simulink model "finalmodel1"  (R2024b)
settings: Solver=FixedStepDiscrete  StartTime=0.0  StopTime=110  FixedStep=SampleTime  MaxStep=1e-3  RelTol=1e-4  AbsTol=1e-3
InitFcn:
  | Ts=50e-6; SampleTime=50e-6; PSSMODEL=1;
  | MB=[1   0.2 30   1.25 40    12 160];
  | 
  | k=[8.3222    2.6014   19.0811    1.9818    3.6841   19.1783  240.6785    2.5684    4.3666   58.7391 7.6960   47.7975    8.7139  296.2463    2.7543    6.5051   47.7755    0.4780   35.4950   18.1866 94.2186]
  | k1=k(1);
  | k2=k(2);
  | k3=k(3);
  | k4=k(4);
  | k5=k(5);
  | k6=k(6);
  | k7=k(7);
  | k8=k(8);
  | k9=k(9);
  | k10=k(10);
  | k11=k(11);
  | k12=k(12);
  | k13=k(13);
  | k14=k(14);
  | k15=k(15);
  | k16=k(16);
  | k17=k(17);
  | k18=k(18);
  | k19=k(19);
  | k20=k(20);
  | k21=k(21);
undefined symbols (not defined in the file or in its folder): dEgdT, DiscIntNeverNeededParam, EgRef, gcbh, Rsh_array5pc, sigbuilder_block, sps_rtmsupport, Tref_K, VT_ref
libraries: spsThreePhaseVIMeasurementLib x14, spsLoadFlowBusLib x9, spsThreePhasePISectionLineLib x6, spsSeriesRLCBranchLib x5, spsThreePhaseTransformerTwoWindingsLib x4, slpidlib x4, spsThreePhaseParallelRLCLoadLib x4, spsThreePhaseSeriesRLCBranchLib x3, spsAlphaBetaZerotodq0Lib x2, spsSynchronousMachinepuStandardLib x2, spsExcitationSystemLib x2, spsMultiBandPowerSystemStabilizerLib x2
(part 8 of 9)

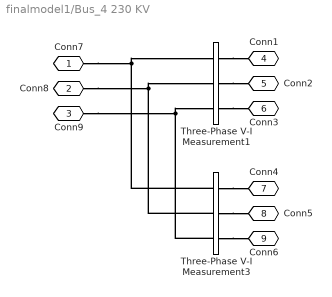
== system finalmodel1/Bus_4 230 KV ==
  Three-Phase V-I Measurement1 : spsThreePhaseVIMeasurementLib/Three-Phase V-I Measurement  VoltageMeasurement=phase-to-ground  SetLabelV=on  LabelV=Vabc_45  Vpu=on  VpuLL=off  CurrentMeasurement=yes  SetLabelI=on  LabelI=Iabc_45  Ipu=on  Pbase=100e6  Vbase=230e3  OutputType=Complex  PhasorSimulation=off  PSBequivalent=0
  Three-Phase V-I Measurement3 : spsThreePhaseVIMeasurementLib/Three-Phase V-I Measurement  VoltageMeasurement=phase-to-ground  SetLabelV=on  LabelV=Vabc_46  Vpu=on  VpuLL=off  CurrentMeasurement=yes  SetLabelI=on  LabelI=Iabc_46  Ipu=on  Pbase=100e6  Vbase=230e3  OutputType=Complex  PhasorSimulation=off  PSBequivalent=0
  Conn7 : PMIOPort  Side=Left  SampleTime=SampleTime
  Conn8 : PMIOPort  Port=2  Side=Left  SampleTime=SampleTime
  Conn9 : PMIOPort  Port=3  Side=Left  SampleTime=SampleTime
  Conn1 : PMIOPort  Port=4  Side=Right  SampleTime=SampleTime
  Conn2 : PMIOPort  Port=5  Side=Right  SampleTime=SampleTime
  Conn3 : PMIOPort  Port=6  Side=Right  SampleTime=SampleTime
  Conn4 : PMIOPort  Port=7  Side=Right  SampleTime=SampleTime
  Conn5 : PMIOPort  Port=8  Side=Right  SampleTime=SampleTime
  Conn6 : PMIOPort  Port=9  Side=Right  SampleTime=SampleTime
  connections:
  Three-Phase V-I Measurement3/LConn3 -- Conn9/RConn1 -- Three-Phase V-I Measurement1/LConn3
  Three-Phase V-I Measurement3/LConn2 -- Conn8/RConn1 -- Three-Phase V-I Measurement1/LConn2
  Three-Phase V-I Measurement3/LConn1 -- Conn7/RConn1 -- Three-Phase V-I Measurement1/LConn1
  Three-Phase V-I Measurement3/RConn3 -- Conn6/RConn1
  Three-Phase V-I Measurement1/RConn3 -- Conn3/RConn1
  Three-Phase V-I Measurement1/RConn1 -- Conn1/RConn1
  Three-Phase V-I Measurement1/RConn2 -- Conn2/RConn1
  Three-Phase V-I Measurement3/RConn1 -- Conn4/RConn1
  Three-Phase V-I Measurement3/RConn2 -- Conn5/RConn1

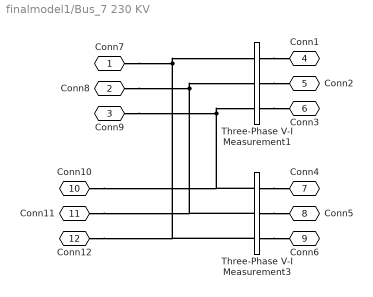
== system finalmodel1/Bus_7 230 KV ==
  Three-Phase V-I Measurement1 : spsThreePhaseVIMeasurementLib/Three-Phase V-I Measurement  VoltageMeasurement=phase-to-ground  SetLabelV=on  LabelV=Vabc_7  Vpu=on  VpuLL=off  CurrentMeasurement=yes  SetLabelI=on  LabelI=Iabc_7  Ipu=on  Pbase=100e6  Vbase=230e3  OutputType=Complex  PhasorSimulation=off  PSBequivalent=0
  Three-Phase V-I Measurement3 : spsThreePhaseVIMeasurementLib/Three-Phase V-I Measurement  VoltageMeasurement=phase-to-ground  SetLabelV=on  LabelV=Vab  Vpu=on  VpuLL=off  CurrentMeasurement=yes  SetLabelI=on  LabelI=Iab  Ipu=on  Pbase=100e6  Vbase=230e3  OutputType=Complex  PhasorSimulation=off  PSBequivalent=0
  Conn7 : PMIOPort  Side=Left  SampleTime=SampleTime
  Conn8 : PMIOPort  Port=2  Side=Left  SampleTime=SampleTime
  Conn9 : PMIOPort  Port=3  Side=Left  SampleTime=SampleTime
  Conn1 : PMIOPort  Port=4  Side=Right  SampleTime=SampleTime
  Conn2 : PMIOPort  Port=5  Side=Right  SampleTime=SampleTime
  Conn3 : PMIOPort  Port=6  Side=Right  SampleTime=SampleTime
  Conn4 : PMIOPort  Port=7  Side=Right  SampleTime=SampleTime
  Conn5 : PMIOPort  Port=8  Side=Right  SampleTime=SampleTime
  Conn6 : PMIOPort  Port=9  Side=Right  SampleTime=SampleTime
  Conn10 : PMIOPort  Port=10  Side=Left  SampleTime=SampleTime
  Conn11 : PMIOPort  Port=11  Side=Left  SampleTime=SampleTime
  Conn12 : PMIOPort  Port=12  Side=Left  SampleTime=SampleTime
  connections:
  Three-Phase V-I Measurement3/RConn2 -- Conn5/RConn1
  Three-Phase V-I Measurement3/RConn1 -- Conn4/RConn1
  Three-Phase V-I Measurement1/RConn2 -- Conn2/RConn1
  Three-Phase V-I Measurement1/RConn1 -- Conn1/RConn1
  Three-Phase V-I Measurement1/RConn3 -- Conn3/RConn1
  Three-Phase V-I Measurement3/RConn3 -- Conn6/RConn1
  Conn7/RConn1 -- Three-Phase V-I Measurement3/LConn3 -- Conn12/RConn1 -- Three-Phase V-I Measurement1/LConn1
  Conn8/RConn1 -- Three-Phase V-I Measurement3/LConn2 -- Conn11/RConn1 -- Three-Phase V-I Measurement1/LConn2
  Conn9/RConn1 -- Conn10/RConn1 -- Three-Phase V-I Measurement3/LConn1 -- Three-Phase V-I Measurement1/LConn3

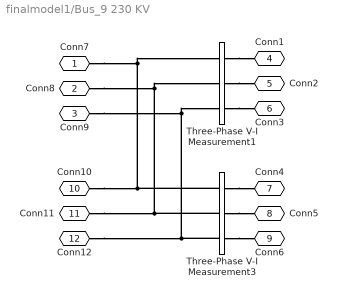
== system finalmodel1/Bus_9 230 KV ==
  Three-Phase V-I Measurement1 : spsThreePhaseVIMeasurementLib/Three-Phase V-I Measurement  VoltageMeasurement=phase-to-ground  SetLabelV=on  LabelV=Vabc_9  Vpu=on  VpuLL=off  CurrentMeasurement=yes  SetLabelI=on  LabelI=Iabc_9  Ipu=on  Pbase=100e6  Vbase=230e3  OutputType=Complex  PhasorSimulation=off  PSBequivalent=0
  Three-Phase V-I Measurement3 : spsThreePhaseVIMeasurementLib/Three-Phase V-I Measurement  VoltageMeasurement=phase-to-ground  SetLabelV=on  LabelV=Vabc  Vpu=on  VpuLL=off  CurrentMeasurement=yes  SetLabelI=on  LabelI=Iabc  Ipu=on  Pbase=100e6  Vbase=230e3  OutputType=Complex  PhasorSimulation=off  PSBequivalent=0
  Conn7 : PMIOPort  Side=Left  SampleTime=SampleTime
  Conn8 : PMIOPort  Port=2  Side=Left  SampleTime=SampleTime
  Conn9 : PMIOPort  Port=3  Side=Left  SampleTime=SampleTime
  Conn1 : PMIOPort  Port=4  Side=Right  SampleTime=SampleTime
  Conn2 : PMIOPort  Port=5  Side=Right  SampleTime=SampleTime
  Conn3 : PMIOPort  Port=6  Side=Right  SampleTime=SampleTime
  Conn4 : PMIOPort  Port=7  Side=Right  SampleTime=SampleTime
  Conn5 : PMIOPort  Port=8  Side=Right  SampleTime=SampleTime
  Conn6 : PMIOPort  Port=9  Side=Right  SampleTime=SampleTime
  Conn10 : PMIOPort  Port=10  Side=Left  SampleTime=SampleTime
  Conn11 : PMIOPort  Port=11  Side=Left  SampleTime=SampleTime
  Conn12 : PMIOPort  Port=12  Side=Left  SampleTime=SampleTime
  connections:
  Conn12/RConn1 -- Three-Phase V-I Measurement3/LConn3 -- Conn9/RConn1 -- Three-Phase V-I Measurement1/LConn3
  Conn11/RConn1 -- Three-Phase V-I Measurement3/LConn2 -- Conn8/RConn1 -- Three-Phase V-I Measurement1/LConn2
  Conn10/RConn1 -- Three-Phase V-I Measurement3/LConn1 -- Conn7/RConn1 -- Three-Phase V-I Measurement1/LConn1
  Three-Phase V-I Measurement3/RConn3 -- Conn6/RConn1
  Three-Phase V-I Measurement1/RConn3 -- Conn3/RConn1
  Three-Phase V-I Measurement1/RConn1 -- Conn1/RConn1
  Three-Phase V-I Measurement1/RConn2 -- Conn2/RConn1
  Three-Phase V-I Measurement3/RConn1 -- Conn4/RConn1
  Three-Phase V-I Measurement3/RConn2 -- Conn5/RConn1

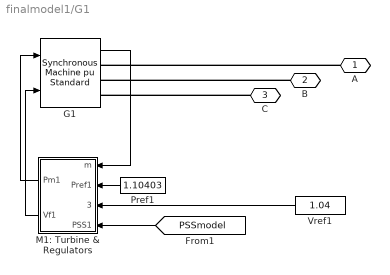
== system finalmodel1/G1 ==
  G1 : spsSynchronousMachinepuStandardLib/Synchronous Machine pu Standard  PresetModel=No  MechanicalLoad=Mechanical power Pm  ShowDetailedParameters=on  RotorType=Round  Units=per unit standard parameters  MeasurementBus=off  NominalParameters="[247.5e6  16500   60 ]"  Reactances1=[1.146 0.2998 0.25 0.969 0.45 0.25 0.025]  Reactances2=[ 1.305, 0.296, 0.252, 0.474, 0.243, 0.18 ]  dAxisTimeConstants=Open-circuit  qAxisTimeConstants=Open-circuit  TimeConstants1=[]  TimeConstants2=[8.96 0.05 0.31 0.05]  TimeConstants3=[]  TimeConstants4=[]  TimeConstants5=[ 1.01, 0.053, 0.1 ]  TimeConstants6=[]  TimeConstants7=[]  TimeConstants8=[]  StatorResistance=0.0025  Mechanical="[ 23.64  0  4]"  PolePairs=4  InitialConditions=[0 -52.9545 0.924925 0.924925 0.924925 -8.45401 -128.454 111.546 1.58772]  SetSaturation=off  Saturation=[0.6404,0.7127,0.8441,0.9214,0.9956,1.082,1.19,1.316,1.457;0.7,0.7698,0.8872,0.9466,0.9969,1.046,1.1,1.151,1.201]  LoadFlowParameters=[2 128000000 0 0 0]  TsPowergui=0  TsBlock=-1  IterativeModel=Trapezoidal non iterative  IterativeDiscreteModel=Trapezoidal non iterative  BusType=swing  Pref=NaN  Qref=0  Qmin=-Inf  Qmax=Inf  PLF=0  QLF=0
      link override Electrical model/Synchronous Machine Discrete Model/Saturation/Lmd_sat/Lmd_sat: SampleTime=SampleTime
      link override Electrical model/Synchronous Machine Discrete Model/Saturation/Lmq_sat/Lmq_sat: SampleTime=SampleTime
      link override Electrical model/Synchronous Machine Discrete Model/phi/Digital Clock: SampleTime=SampleTime
      link override Electrical model/Synchronous Machine Discrete Model/phi/fluxes: SampleTime=SampleTime
      link override Electrical model/Synchronous Machine Discrete Model/phi/voltages: SampleTime=SampleTime
      link override Mechanical model/Delay Prediction/dw_delay: SampleTime=SampleTime
      link override Mechanical model/Delay Prediction/dw_predict: SampleTime=SampleTime
      link override Mechanical model/Digital Clock: SampleTime=SampleTime
      link override Mechanical model/Fcn: Expr=rem(u,2*pi)
      link override Mechanical model/Rotor angle dthetae: SampleTime=SampleTime
      link override Mechanical model/Rotor speed deviation (dw): SampleTime=SampleTime
      link override Mechanical model/theta: SampleTime=SampleTime
  M1: Turbine & Regulators : Subsystem
  Pref1 : Constant  Value=1.10403  SampleTime=SampleTime
  Vref1 : Constant  Value=1.04  SampleTime=SampleTime
  A : PMIOPort  Side=Left  SampleTime=SampleTime
  B : PMIOPort  Port=2  Side=Left  SampleTime=SampleTime
  C : PMIOPort  Port=3  Side=Left  SampleTime=SampleTime
  wires:
  Pref1/1 -> M1: Turbine & Regulators/2(Pref1)
  [PSSmodel] -> M1: Turbine & Regulators/4(PSS1)
  M1: Turbine & Regulators/1(Pm1) -> G1/1
  M1: Turbine & Regulators/2(Vf1) -> G1/2
  G1/1 -> M1: Turbine & Regulators/1(m)
  Vref1/1 -> M1: Turbine & Regulators/3(Vref1)
  connections:
  A/RConn1 -- G1/RConn1
  B/RConn1 -- G1/RConn2
  C/RConn1 -- G1/RConn3

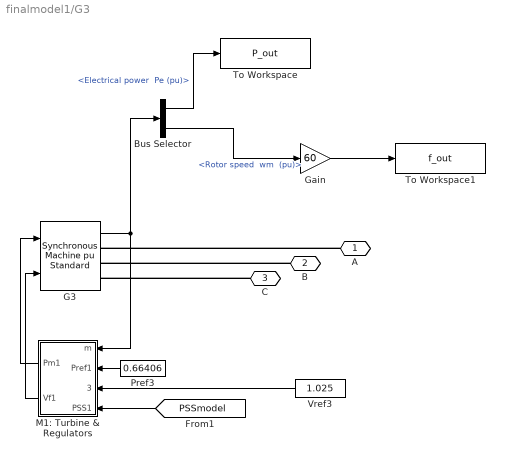
== system finalmodel1/G3 ==
  Bus Selector : BusSelector  OutputSignals="Mechanical.Electrical power  Pe (pu),Mechanical.Rotor speed  wm  (pu)"
  G3 : spsSynchronousMachinepuStandardLib/Synchronous Machine pu Standard  PresetModel=No  MechanicalLoad=Mechanical power Pm  ShowDetailedParameters=on  RotorType=Round  Units=per unit standard parameters  MeasurementBus=off  NominalParameters="[128e6  13800   60 ]"  Reactances1=[1.3125 0.2998 0.25 1.2578 0.45 0.25 0.025]  Reactances2=[ 1.305, 0.296, 0.252, 0.474, 0.243, 0.18 ]  dAxisTimeConstants=Open-circuit  qAxisTimeConstants=Open-circuit  TimeConstants1=[]  TimeConstants2=[5.89 0.05 0.6 0.05]  TimeConstants3=[]  TimeConstants4=[]  TimeConstants5=[ 1.01, 0.053, 0.1 ]  TimeConstants6=[]  TimeConstants7=[]  TimeConstants8=[]  StatorResistance=0.0025  Mechanical="[ 3.01  0  4]"  PolePairs=4  InitialConditions=[0 -58.3097 0.651492 0.651492 0.651492 -3.18103 -123.181 116.819 1.26474]  SetSaturation=off  Saturation=[0.6404,0.7127,0.8441,0.9214,0.9956,1.082,1.19,1.316,1.457;0.7,0.7698,0.8872,0.9466,0.9969,1.046,1.1,1.151,1.201]  LoadFlowParameters=[1 85000000 0 0 0]  TsPowergui=0  TsBlock=-1  IterativeModel=Trapezoidal non iterative  IterativeDiscreteModel=Trapezoidal non iterative  BusType=PV  Pref=85e6  Qref=0  Qmin=-Inf  Qmax=Inf  PLF=0  QLF=0
      link override Electrical model/Synchronous Machine Discrete Model/Saturation/Lmd_sat/Lmd_sat: SampleTime=SampleTime
      link override Electrical model/Synchronous Machine Discrete Model/Saturation/Lmq_sat/Lmq_sat: SampleTime=SampleTime
      link override Electrical model/Synchronous Machine Discrete Model/phi/Digital Clock: SampleTime=SampleTime
      link override Electrical model/Synchronous Machine Discrete Model/phi/fluxes: SampleTime=SampleTime
      link override Electrical model/Synchronous Machine Discrete Model/phi/voltages: SampleTime=SampleTime
      link override Mechanical model/Delay Prediction/dw_delay: SampleTime=SampleTime
      link override Mechanical model/Delay Prediction/dw_predict: SampleTime=SampleTime
      link override Mechanical model/Digital Clock: SampleTime=SampleTime
      link override Mechanical model/Fcn: Expr=rem(u,2*pi)
      link override Mechanical model/Rotor angle dthetae: SampleTime=SampleTime
      link override Mechanical model/Rotor speed deviation (dw): SampleTime=SampleTime
      link override Mechanical model/theta: SampleTime=SampleTime
  Gain : Gain  Gain=60  SampleTime=SampleTime
  M1: Turbine & Regulators : Subsystem
  Pref3 : Constant  Value=0.66406  SampleTime=SampleTime
  To Workspace : ToWorkspace  VariableName=P_out  SaveFormat=Timeseries  SampleTime=SampleTime
  To Workspace1 : ToWorkspace  VariableName=f_out  SaveFormat=Timeseries  SampleTime=SampleTime
  Vref3 : Constant  Value=1.025  SampleTime=SampleTime
  A : PMIOPort  Side=Left  SampleTime=SampleTime
  B : PMIOPort  Port=2  Side=Left  SampleTime=SampleTime
  C : PMIOPort  Port=3  Side=Left  SampleTime=SampleTime
  wires:
  Vref3/1 -> M1: Turbine & Regulators/3(Vref1)
  G3/1 -> Bus Selector/1, M1: Turbine & Regulators/1(m)
  M1: Turbine & Regulators/2(Vf1) -> G3/2
  M1: Turbine & Regulators/1(Pm1) -> G3/1
  [PSSmodel] -> M1: Turbine & Regulators/4(PSS1)
  Pref3/1 -> M1: Turbine & Regulators/2(Pref1)
  Gain/1 -> To Workspace1/1
  Bus Selector/1 -> To Workspace/1  "<Electrical power  Pe (pu)>"
  Bus Selector/2 -> Gain/1  "<Rotor speed  wm  (pu)>"
  connections:
  C/RConn1 -- G3/RConn3
  B/RConn1 -- G3/RConn2
  A/RConn1 -- G3/RConn1

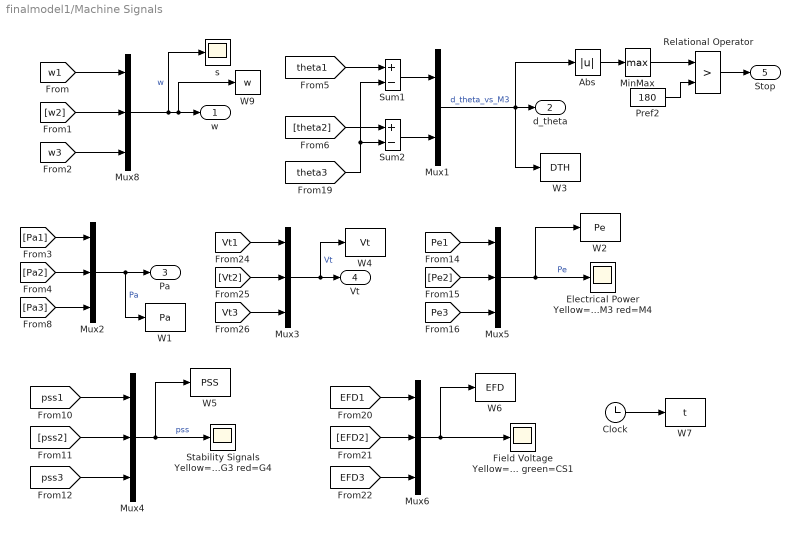
== system finalmodel1/Machine Signals ==
  Abs : Abs  SampleTime=SampleTime
  Clock : Clock
  "Electrical Power Yellow=M1 mag=M2 cyan=M3 red=M4 " : Scope
  Field Voltage Yellow=G1 mag=G2 cyan=G3 red=G4 green=CS1 : Scope
  MinMax : MinMax  Function=max  InputSameDT=on  SaturateOnIntegerOverflow=on  SampleTime=SampleTime
  Mux1 : Mux  Inputs=2
  Mux{2..6,8} (6 alike) : Mux  Inputs=3
  Pref2 : Constant  Value=180  SampleTime=SampleTime
  Relational Operator : RelationalOperator  Operator=>  SampleTime=SampleTime
  "Stability Signals Yellow=G1 mag=G2 cyan=G3 red=G4 " : Scope
  Sum1 : Sum  Inputs=+-  InputSameDT=on  SaturateOnIntegerOverflow=on  SampleTime=SampleTime  OutDataTypeStr=Inherit: Same as first input
  Sum2 : Sum  Inputs=+-  InputSameDT=on  SaturateOnIntegerOverflow=on  SampleTime=SampleTime  OutDataTypeStr=Inherit: Same as first input
  W1 : ToWorkspace  VariableName=Pa  SaveFormat=Timeseries  SampleTime=SampleTime
  W2 : ToWorkspace  VariableName=Pe  SaveFormat=Timeseries  SampleTime=SampleTime
  W3 : ToWorkspace  VariableName=DTH  SaveFormat=Timeseries  SampleTime=SampleTime
  W4 : ToWorkspace  VariableName=Vt  SaveFormat=Timeseries  SampleTime=SampleTime
  W5 : ToWorkspace  VariableName=PSS  SaveFormat=Timeseries  SampleTime=SampleTime
  W6 : ToWorkspace  VariableName=EFD  SaveFormat=Timeseries  SampleTime=SampleTime
  W7 : ToWorkspace  VariableName=t  SaveFormat=Timeseries  SampleTime=SampleTime
  W9 : ToWorkspace  VariableName=w  SaveFormat=Timeseries  SampleTime=SampleTime
  s : Scope
  w : Outport  SampleTime=SampleTime
  d_theta : Outport  Port=2  SampleTime=SampleTime
  Pa : Outport  Port=3  SampleTime=SampleTime
  Vt : Outport  Port=4  SampleTime=SampleTime
  Stop : Outport  Port=5  SampleTime=SampleTime
  wires:
  Mux8/1 -> s/1, W9/1, w/1  "w"
  [w1] -> Mux8/1
  [w2] -> Mux8/2
  [w3] -> Mux8/3
  Mux1/1 -> d_theta/1, Abs/1, W3/1  "d_theta_vs_M3"
  Abs/1 -> MinMax/1
  Pref2/1 -> Relational Operator/2
  MinMax/1 -> Relational Operator/1
  [Pa1] -> Mux2/1
  Mux4/1 -> "Stability Signals Yellow=G1 mag=G2 cyan=G3 red=G4 "/1, W5/1  "pss"
  [pss1] -> Mux4/1
  [pss2] -> Mux4/2
  [pss3] -> Mux4/3
  [EFD1] -> Mux6/1
  [EFD2] -> Mux6/2
  [EFD3] -> Mux6/3
  Mux6/1 -> Field Voltage Yellow=G1 mag=G2 cyan=G3 red=G4 green=CS1/1, W6/1
  Relational Operator/1 -> Stop/1
  Mux2/1 -> Pa/1, W1/1  "Pa"
  [theta1] -> Sum1/1
  Sum1/1 -> Mux1/1
  [theta2] -> Sum2/1
  [theta3] -> Sum1/2, Sum2/2
  Sum2/1 -> Mux1/2
  [Pa2] -> Mux2/2
  [Pa3] -> Mux2/3
  [Vt1] -> Mux3/1
  [Vt2] -> Mux3/2
  [Vt3] -> Mux3/3
  Mux3/1 -> Vt/1, W4/1  "Vt"
  [Pe1] -> Mux5/1
  [Pe2] -> Mux5/2
  [Pe3] -> Mux5/3
  Mux5/1 -> "Electrical Power Yellow=M1 mag=M2 cyan=M3 red=M4 "/1, W2/1  "Pe"
  Clock/1 -> W7/1

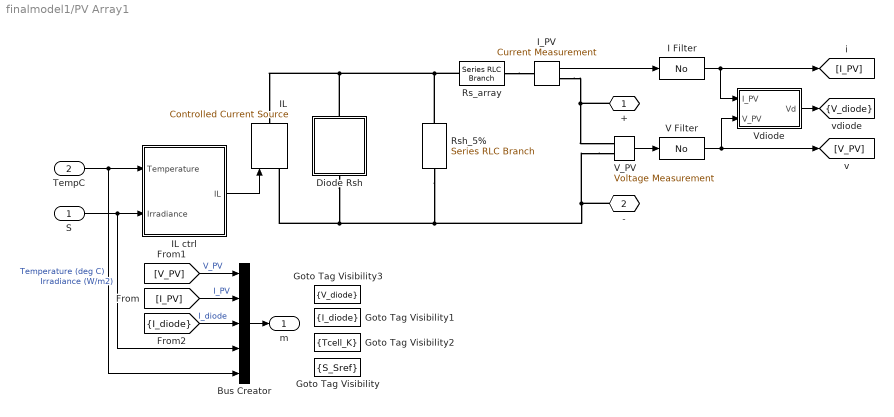
== system finalmodel1/PV Array1 ==
  S : Inport
  TempC : Inport  Port=2
  Bus Creator : BusCreator  Inputs=5
  Diode Rsh : Subsystem
      mask Display:
      | plot(-75,-50,100,150, [-15 -15 43 -15 -15 -75],[50 8 50 92 50 50], ...
      |     [43 43],[8 94],[100 43], [50 50])
  Goto Tag Visibility : GotoTagVisibility  GotoTag=S_Sref
  Goto Tag Visibility1 : GotoTagVisibility  GotoTag=I_diode
  Goto Tag Visibility2 : GotoTagVisibility  GotoTag=Tcell_K
  Goto Tag Visibility3 : GotoTagVisibility  GotoTag=V_diode
  I Filter : spsPVarrayModel/No  SystemSampleTime=-1  VariantControl=Variant1  VariantActivationTime=update diagram  AllowFlexibleInterface=on  Latency=0  AutoFrameSizeCalculation=off
  IL : spsControlledCurrentSourceLib/Controlled Current Source  Initialize=on  Source_Type=AC  Amplitude=0  Phase=0  Frequency=0  Measurements=None
  IL ctrl : Subsystem
  I_PV : spsCurrentMeasurementLib/Current Measurement  PhasorSimulation=off  OutputType=Complex  PSBequivalent=0
  Rs_array : spsSeriesRLCBranchLib/Series RLC Branch  LConnTagsString=__new0  RConnTagsString=__new0  BranchType=R  Resistance=Rs*Nser/Npar  Inductance=1e-3  SetiL0=off  InitialCurrent=0  Capacitance=1e-6  Setx0=off  InitialVoltage=0  Measurements=None
  Rsh_5% : spsSeriesRLCBranchLib/Series RLC Branch  LConnTagsString=__new0  RConnTagsString=__new0  BranchType=R  Resistance=Rsh_array5pc  Inductance=1e-3  SetiL0=off  InitialCurrent=0  Capacitance=1e-6  Setx0=off  InitialVoltage=0  Measurements=None
  V Filter : spsPVarrayModel/No  SystemSampleTime=-1  VariantControl=Variant1  VariantActivationTime=update diagram  AllowFlexibleInterface=on  Latency=0  AutoFrameSizeCalculation=off
  V_PV : spsVoltageMeasurementLib/Voltage Measurement  PhasorSimulation=off  OutputType=Complex  PSBequivalent=0
  Vdiode : Subsystem
  + : PMIOPort  Side=Right
  - : PMIOPort  Port=2  Side=Right
  m : Outport  VectorParamsAs1DForOutWhenUnconnected=off
  tag scope: V_diode=scoped
  wires:
  TempC/1 -> Bus Creator/5, IL ctrl/1(Temperature)  "Temperature (deg C)"
  S/1 -> IL ctrl/2(Irradiance), Bus Creator/4  "Irradiance (W/m2)"
  I_PV/1 -> I Filter/1
  Bus Creator/1 -> m/1
  IL ctrl/1(IL) -> IL/1
  V_PV/1 -> V Filter/1
  I Filter/1 -> Vdiode/1(I_PV), [I_PV]
  V Filter/1 -> [V_PV], Vdiode/2(V_PV)
  [I_PV] -> Bus Creator/2  "I_PV"
  [V_PV] -> Bus Creator/1  "V_PV"
  [I_diode] -> Bus Creator/3  "I_diode"
  Vdiode/1(Vd) -> [V_diode]
  connections:
  +/RConn1 -- I_PV/RConn1 -- V_PV/LConn1
  Rs_array/LConn1 -- Rsh_5%/LConn1 -- Diode Rsh/LConn1 -- IL/RConn1
  V_PV/LConn2 -- Diode Rsh/RConn1 -- IL/LConn1 -- Rsh_5%/RConn1 -- -/RConn1
  Rs_array/RConn1 -- I_PV/LConn1

== system finalmodel1/Signal Builder2 ==
  Demux : Demux  Tag=STV Demux  Outputs=1
      settings: DisplayOption=none
  FromWs : FromWorkspace  Tag=STV FromWs  VariableName=tuvar
      SigBuilderData=|
      | common.afterFinalStr = 'Extrapolate'
      | common.sampleTime = 0
      | dataSet.timeRange = [0 4]
      | dataSet.name = 'Group 1'
      | sbobj.Groups.Name = 'Group 1'
      | sbobj.Groups.Signals.Name = 'Signal 1'
      | sbobj.Groups.Signals.XData = [0 0.00416233090531 0.00832466181061 0.0124869927159 0.0166493236212 0.0208116545265 0.0249739854318 0.0291363163371 0.0332986472425 0.0374609781478 0.0416233090531 0.0457856399584 ... (962 elements, 1x962)]
      | sbobj.Groups.Signals.YData = [2.47122187864 2.47122187864 2.47122187864 2.47122187864 2.47122187864 2.47122187864 2.47122187864 2.47122187864 2.47122187864 2.47121149505 2.47121149505 2.47121149505 ... (962 elements, 1x962)]
      | sbobj.Groups.TimeRange = [0 4]
  Signal 1 : Outport  Tag=STV Outport  VectorParamsAs1DForOutWhenUnconnected=off
  wires:
  FromWs/1 -> Demux/1
  Demux/1 -> Signal 1/1

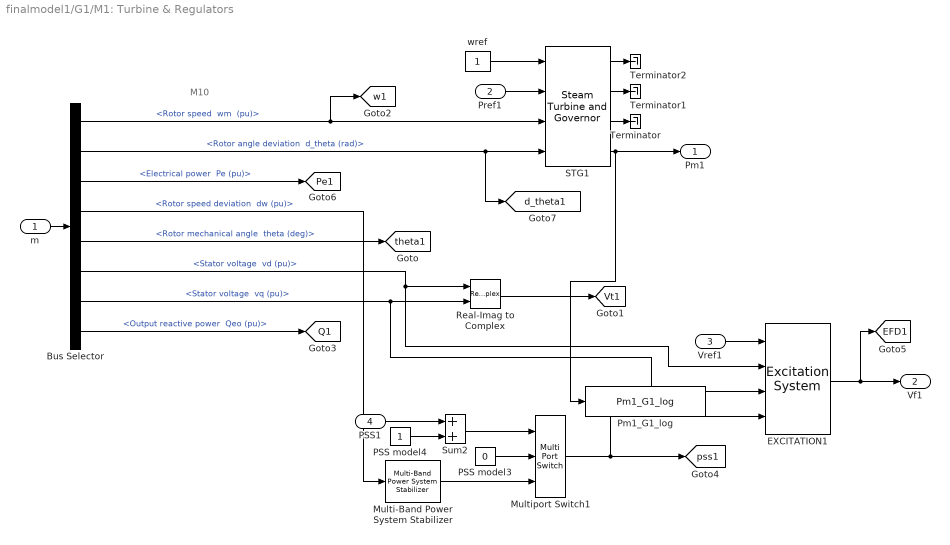
== system finalmodel1/G1/M1: Turbine & Regulators ==
  note: M10
  m : Inport  SampleTime=SampleTime
  Pref1 : Inport  Port=2  SampleTime=SampleTime
  Vref1 : Inport  Port=3  SampleTime=SampleTime
  PSS1 : Inport  Port=4  SampleTime=SampleTime
  Bus Selector : BusSelector  OutputSignals="Mechanical.Rotor speed  wm  (pu),Mechanical.Rotor angle deviation  d_theta (rad),Mechanical.Electrical power  Pe (pu),Mechanical.Rotor speed deviation  dw (pu),Mechanical.Rotor mechanical angle  theta (deg),dq0 components.Stator voltage  vd (pu),dq0 components.Stator voltage  vq (pu),Output reactive power  Qeo (pu)"
  EXCITATION1 : spsExcitationSystemLib/Excitation System  tr=0.01  reg=[20 0.2 ]  exc=[ 1, 0.314 ]  tgr=[10 1]  damp=[ 0, 0 ]  sat=[ 0, 0 ]  lim="[-5 5  0 ]"  v0=[1.04 1.5877]
      link override Model: Ts=SampleTime
      link override Model/Damping kfd.s // (tfd.s +1)/1st-Order Discrete Filter: Ts=SampleTime
      link override Model/Damping kfd.s // (tfd.s +1)/1st-Order Discrete Filter/Discrete State-Space: SampleTime=SampleTime
      link override Model/Exciter  1 // (te.s + ke)/1st order Lowpass: Ts=SampleTime
      link override Model/Exciter  1 // (te.s + ke)/1st order Lowpass/Discrete State-Space: SampleTime=SampleTime
      link override Model/Lead Lag Compensator tc.s+1 // tb.s+1: Ts=SampleTime
      link override Model/Lead Lag Compensator tc.s+1 // tb.s+1/Discrete State-Space: SampleTime=SampleTime
      link override Model/Low Pass Filter 1 // (tr.s +1) (with IC): Ts=SampleTime
      link override Model/Low Pass Filter 1 // (tr.s +1) (with IC)/Discrete State-Space: SampleTime=SampleTime
      link override Model/Main Regulator ka // (ta.s +1)/1st order Lowpass: Ts=SampleTime
      link override Model/Main Regulator ka // (ta.s +1)/1st order Lowpass/Discrete State-Space: SampleTime=SampleTime
      link override Model/Positive Sequence Voltage: Expr=sqrt(abs(u(1)^2 + u(2)^2))
      link override Model/Unit Delay1: SampleTime=SampleTime
      link override Model/Unit Delay2: SampleTime=SampleTime
      settings: LibrarySourceBlock=sps_lib/Electrical Machines/Synchronous Machine Control/Excitation System
  Multi-Band Power System Stabilizer : spsMultiBandPowerSystemStabilizerLib/Multi-Band Power System Stabilizer  OperationMode=Simplified settings  Kg=k8  GL=[k9 k10]  GI=[k11 k12]  GH=[k13 k14]  GLd=[66 66 9.4]  TcLF=[1.667 2 0 0 0 0 2 2.4 0 0 0 0 1 1]  GId=[66 66 47.6]  TcIF=[1 1 0.25 0.3 0 0 1 1 0.3 0.36 0 0 0 0]  GHd=[66 66 233]  TcHF="[0.01 0.012 0 0 0 0  0.012 0.0144 0 0 0 0 1 1]"  LIM=[.075 .15 .15 .15]  Plot_On=off  MagdB_On=off  FreqRange=logspace(-2,2,500)
      link override Model/Discrete Lead-Lag1: Ts=SampleTime
      link override Model/Discrete Lead-Lag1/Discrete State-Space: SampleTime=SampleTime
      link override Model/Discrete Lead-Lag2: Ts=SampleTime
      link override Model/Discrete Lead-Lag2/Discrete State-Space: SampleTime=SampleTime
      link override Model/Discrete Lead-Lag3: Ts=SampleTime
      link override Model/Discrete Lead-Lag3/Discrete State-Space: SampleTime=SampleTime
      link override Model/Discrete Lead-Lag4: Ts=SampleTime
      link override Model/Discrete Lead-Lag4/Discrete State-Space: SampleTime=SampleTime
      link override Model/Discrete Lead-Lag5: Ts=SampleTime
      link override Model/Discrete Lead-Lag5/Discrete State-Space: SampleTime=SampleTime
      link override Model/Discrete Lead-Lag6: Ts=SampleTime
      link override Model/Discrete Lead-Lag6/Discrete State-Space: SampleTime=SampleTime
      link override Model/HF speed sensor: Ts=SampleTime
      link override Model/HF speed sensor/Discrete State-Space: SampleTime=SampleTime
      link override Model/LF and IF speed sensor: Ts=SampleTime
      link override Model/LF and IF speed sensor/Discrete State-Space: SampleTime=SampleTime
      link override Model/Transfer function for detailed model (HF)/Transfer functions for detailed stabilizer/Discrete Lead-Lag1: Ts=SampleTime
      link override Model/Transfer function for detailed model (HF)/Transfer functions for detailed stabilizer/Discrete Lead-Lag1/Discrete State-Space: SampleTime=SampleTime
      link override Model/Transfer function for detailed model (HF)/Transfer functions for detailed stabilizer/Discrete Lead-Lag2: Ts=SampleTime
      link override Model/Transfer function for detailed model (HF)/Transfer functions for detailed stabilizer/Discrete Lead-Lag2/Discrete State-Space: SampleTime=SampleTime
      link override Model/Transfer function for detailed model (HF)/Transfer functions for detailed stabilizer1/Discrete Lead-Lag1: Ts=SampleTime
      link override Model/Transfer function for detailed model (HF)/Transfer functions for detailed stabilizer1/Discrete Lead-Lag1/Discrete State-Space: SampleTime=SampleTime
      link override Model/Transfer function for detailed model (HF)/Transfer functions for detailed stabilizer1/Discrete Lead-Lag2: Ts=SampleTime
      link override Model/Transfer function for detailed model (HF)/Transfer functions for detailed stabilizer1/Discrete Lead-Lag2/Discrete State-Space: SampleTime=SampleTime
      link override Model/Transfer function for detailed model (IF)/Transfer functions for detailed stabilizer/Discrete Lead-Lag1: Ts=SampleTime
      link override Model/Transfer function for detailed model (IF)/Transfer functions for detailed stabilizer/Discrete Lead-Lag1/Discrete State-Space: SampleTime=SampleTime
      link override Model/Transfer function for detailed model (IF)/Transfer functions for detailed stabilizer/Discrete Lead-Lag2: Ts=SampleTime
      link override Model/Transfer function for detailed model (IF)/Transfer functions for detailed stabilizer/Discrete Lead-Lag2/Discrete State-Space: SampleTime=SampleTime
      link override Model/Transfer function for detailed model (IF)/Transfer functions for detailed stabilizer1/Discrete Lead-Lag1: Ts=SampleTime
      link override Model/Transfer function for detailed model (IF)/Transfer functions for detailed stabilizer1/Discrete Lead-Lag1/Discrete State-Space: SampleTime=SampleTime
      link override Model/Transfer function for detailed model (IF)/Transfer functions for detailed stabilizer1/Discrete Lead-Lag2: Ts=SampleTime
      link override Model/Transfer function for detailed model (IF)/Transfer functions for detailed stabilizer1/Discrete Lead-Lag2/Discrete State-Space: SampleTime=SampleTime
      link override Model/Transfer function for detailed model (LF)/Transfer functions for detailed stabilizer/Discrete Lead-Lag1: Ts=SampleTime
      link override Model/Transfer function for detailed model (LF)/Transfer functions for detailed stabilizer/Discrete Lead-Lag1/Discrete State-Space: SampleTime=SampleTime
      link override Model/Transfer function for detailed model (LF)/Transfer functions for detailed stabilizer/Discrete Lead-Lag2: Ts=SampleTime
      link override Model/Transfer function for detailed model (LF)/Transfer functions for detailed stabilizer/Discrete Lead-Lag2/Discrete State-Space: SampleTime=SampleTime
      link override Model/Transfer function for detailed model (LF)/Transfer functions for detailed stabilizer1/Discrete Lead-Lag1: Ts=SampleTime
      link override Model/Transfer function for detailed model (LF)/Transfer functions for detailed stabilizer1/Discrete Lead-Lag1/Discrete State-Space: SampleTime=SampleTime
      link override Model/Transfer function for detailed model (LF)/Transfer functions for detailed stabilizer1/Discrete Lead-Lag2: Ts=SampleTime
      link override Model/Transfer function for detailed model (LF)/Transfer functions for detailed stabilizer1/Discrete Lead-Lag2/Discrete State-Space: SampleTime=SampleTime
      settings: LibrarySourceBlock=|
      | sps_lib/Electrical Machines/Synchronous Machine Control/Multi-Band
      | Power System Stabilizer
  Multiport Switch1 : MultiPortSwitch  Inputs=2  SampleTime=SampleTime  SaturateOnIntegerOverflow=off
  PSS model3 : Constant  Value=0  SampleTime=SampleTime
  PSS model4 : Constant  SampleTime=SampleTime
  Pm1_G1_log : ToWorkspace  VariableName=Pm1_G1_log  SaveFormat=Timeseries  SampleTime=-1
  Real-Imag to Complex : RealImagToComplex  SampleTime=SampleTime
  STG1 : spsSteamTurbineandGovernorLib/Steam Turbine and Governor  gentype=Tandem-compound (single mass)  reg1="[ 1  0.05    0 ]"  reg2="[ 0.001  0.15 ]"  reg3="[ -0.1  0.1  0  4.496 ]"  N=3600  turb1="[ 0  10   3.3   0.5   ]"  turb2="[   0   0.36    0.36   0.28   ]"  HA="[ 0.046  1.430  1.465   0.192 ]"  KA="[ 90.44  53.88  64.59   62.94  ]"  DA="[ 0.0115  0.3575  0.3663   0.0137  ]"  ini1=0.95361  ini2=[0.779316,-31.4247]
      link override Model/4 mass shaft/1 mass/Mass2: Ts=SampleTime
      link override Model/4 mass shaft/1 mass/Mass2/Ad*x(k-1): SampleTime=SampleTime
      link override Model/4 mass shaft/1 mass/Mass2/Bd*(u(k)+ u(k-1)): SampleTime=SampleTime
      link override Model/4 mass shaft/1 mass/Mass2/Delay_u: SampleTime=SampleTime
      link override Model/4 mass shaft/1 mass/Mass2/Delay_x: SampleTime=SampleTime
      link override Model/4 mass shaft/1 mass/Mass2/Digital Clock: SampleTime=SampleTime
      link override Model/4 mass shaft/1 mass/Mass2/Prediction/Unit Delay3: SampleTime=SampleTime
      link override Model/4 mass shaft/2 masses/Mass2: Ts=SampleTime
      link override Model/4 mass shaft/2 masses/Mass2/Ad*x(k-1): SampleTime=SampleTime
      link override Model/4 mass shaft/2 masses/Mass2/Bd*(u(k)+ u(k-1)): SampleTime=SampleTime
      link override Model/4 mass shaft/2 masses/Mass2/Delay_u: SampleTime=SampleTime
      link override Model/4 mass shaft/2 masses/Mass2/Delay_x: SampleTime=SampleTime
      link override Model/4 mass shaft/2 masses/Mass2/Digital Clock: SampleTime=SampleTime
      link override Model/4 mass shaft/2 masses/Mass2/Prediction/Unit Delay3: SampleTime=SampleTime
      link override Model/4 mass shaft/2 masses/Mass3: Ts=SampleTime
      link override Model/4 mass shaft/2 masses/Mass3/Ad*x(k-1): SampleTime=SampleTime
      link override Model/4 mass shaft/2 masses/Mass3/Bd*(u(k)+ u(k-1)): SampleTime=SampleTime
      link override Model/4 mass shaft/2 masses/Mass3/Delay_u: SampleTime=SampleTime
      link override Model/4 mass shaft/2 masses/Mass3/Delay_x: SampleTime=SampleTime
      link override Model/4 mass shaft/2 masses/Mass3/Digital Clock: SampleTime=SampleTime
      link override Model/4 mass shaft/2 masses/Mass3/Prediction/Unit Delay3: SampleTime=SampleTime
      link override Model/4 mass shaft/3 masses/Mass2: Ts=SampleTime
      link override Model/4 mass shaft/3 masses/Mass2/Ad*x(k-1): SampleTime=SampleTime
      link override Model/4 mass shaft/3 masses/Mass2/Bd*(u(k)+ u(k-1)): SampleTime=SampleTime
      link override Model/4 mass shaft/3 masses/Mass2/Delay_u: SampleTime=SampleTime
      link override Model/4 mass shaft/3 masses/Mass2/Delay_x: SampleTime=SampleTime
      link override Model/4 mass shaft/3 masses/Mass2/Digital Clock: SampleTime=SampleTime
      link override Model/4 mass shaft/3 masses/Mass2/Prediction/Unit Delay3: SampleTime=SampleTime
      link override Model/4 mass shaft/3 masses/Mass3: Ts=SampleTime
      link override Model/4 mass shaft/3 masses/Mass3/Ad*x(k-1): SampleTime=SampleTime
      link override Model/4 mass shaft/3 masses/Mass3/Bd*(u(k)+ u(k-1)): SampleTime=SampleTime
      link override Model/4 mass shaft/3 masses/Mass3/Delay_u: SampleTime=SampleTime
      link override Model/4 mass shaft/3 masses/Mass3/Delay_x: SampleTime=SampleTime
      link override Model/4 mass shaft/3 masses/Mass3/Digital Clock: SampleTime=SampleTime
      link override Model/4 mass shaft/3 masses/Mass3/Prediction/Unit Delay3: SampleTime=SampleTime
      link override Model/4 mass shaft/3 masses/Mass4: Ts=SampleTime
      link override Model/4 mass shaft/3 masses/Mass4/Ad*x(k-1): SampleTime=SampleTime
      link override Model/4 mass shaft/3 masses/Mass4/Bd*(u(k)+ u(k-1)): SampleTime=SampleTime
      link override Model/4 mass shaft/3 masses/Mass4/Delay_u: SampleTime=SampleTime
      link override Model/4 mass shaft/3 masses/Mass4/Delay_x: SampleTime=SampleTime
      link override Model/4 mass shaft/3 masses/Mass4/Digital Clock: SampleTime=SampleTime
      link override Model/4 mass shaft/3 masses/Mass4/Prediction/Unit Delay3: SampleTime=SampleTime
      link override Model/4 mass shaft/4 masses/Mass2: Ts=SampleTime
      link override Model/4 mass shaft/4 masses/Mass2/Ad*x(k-1): SampleTime=SampleTime
      link override Model/4 mass shaft/4 masses/Mass2/Bd*(u(k)+ u(k-1)): SampleTime=SampleTime
      link override Model/4 mass shaft/4 masses/Mass2/Delay_u: SampleTime=SampleTime
      link override Model/4 mass shaft/4 masses/Mass2/Delay_x: SampleTime=SampleTime
      link override Model/4 mass shaft/4 masses/Mass2/Digital Clock: SampleTime=SampleTime
      link override Model/4 mass shaft/4 masses/Mass2/Prediction/Unit Delay3: SampleTime=SampleTime
      link override Model/4 mass shaft/4 masses/Mass3: Ts=SampleTime
      link override Model/4 mass shaft/4 masses/Mass3/Ad*x(k-1): SampleTime=SampleTime
      link override Model/4 mass shaft/4 masses/Mass3/Bd*(u(k)+ u(k-1)): SampleTime=SampleTime
      link override Model/4 mass shaft/4 masses/Mass3/Delay_u: SampleTime=SampleTime
      link override Model/4 mass shaft/4 masses/Mass3/Delay_x: SampleTime=SampleTime
      link override Model/4 mass shaft/4 masses/Mass3/Digital Clock: SampleTime=SampleTime
      link override Model/4 mass shaft/4 masses/Mass3/Prediction/Unit Delay3: SampleTime=SampleTime
      link override Model/4 mass shaft/4 masses/Mass4: Ts=SampleTime
      link override Model/4 mass shaft/4 masses/Mass4/Ad*x(k-1): SampleTime=SampleTime
      link override Model/4 mass shaft/4 masses/Mass4/Bd*(u(k)+ u(k-1)): SampleTime=SampleTime
      link override Model/4 mass shaft/4 masses/Mass4/Delay_u: SampleTime=SampleTime
      link override Model/4 mass shaft/4 masses/Mass4/Delay_x: SampleTime=SampleTime
      link override Model/4 mass shaft/4 masses/Mass4/Digital Clock: SampleTime=SampleTime
      link override Model/4 mass shaft/4 masses/Mass4/Prediction/Unit Delay3: SampleTime=SampleTime
      link override Model/4 mass shaft/4 masses/Mass5: Ts=SampleTime
      link override Model/4 mass shaft/4 masses/Mass5/Ad*x(k-1): SampleTime=SampleTime
      link override Model/4 mass shaft/4 masses/Mass5/Bd*(u(k)+ u(k-1)): SampleTime=SampleTime
      link override Model/4 mass shaft/4 masses/Mass5/Delay_u: SampleTime=SampleTime
      link override Model/4 mass shaft/4 masses/Mass5/Delay_x: SampleTime=SampleTime
      link override Model/4 mass shaft/4 masses/Mass5/Digital Clock: SampleTime=SampleTime
      link override Model/4 mass shaft/4 masses/Mass5/Prediction/Unit Delay3: SampleTime=SampleTime
      link override Model/speed regulator/Servo-motor Position: SampleTime=SampleTime
      link override Model/speed regulator/Speed Relay: Ts=SampleTime
      link override Model/speed regulator/Speed Relay/In: SampleTime=SampleTime
      link override Model/speed regulator/Speed Relay/Model/Delay_x: SampleTime=SampleTime
      link override Model/speed regulator/Speed Relay/Out: SampleTime=SampleTime
      link override Model/steam turbine/Stage 1/Constant4: SampleTime=SampleTime
      link override Model/steam turbine/Stage 1/Stage1/Stage1: Ts=SampleTime
      link override Model/steam turbine/Stage 1/Stage1/Stage1/In: SampleTime=SampleTime
      link override Model/steam turbine/Stage 1/Stage1/Stage1/Model/Delay_x: SampleTime=SampleTime
      link override Model/steam turbine/Stage 1/Stage1/Stage1/Out: SampleTime=SampleTime
      link override Model/steam turbine/Stage 2 /Constant3: SampleTime=SampleTime
      link override Model/steam turbine/Stage 2 /Stage2/Stage2: Ts=SampleTime
      link override Model/steam turbine/Stage 2 /Stage2/Stage2/In: SampleTime=SampleTime
      link override Model/steam turbine/Stage 2 /Stage2/Stage2/Model/Delay_x: SampleTime=SampleTime
      link override Model/steam turbine/Stage 2 /Stage2/Stage2/Out: SampleTime=SampleTime
      link override Model/steam turbine/Stage 3/Constant2: SampleTime=SampleTime
      link override Model/steam turbine/Stage 3/Stage3/Stage3: Ts=SampleTime
      link override Model/steam turbine/Stage 3/Stage3/Stage3/In: SampleTime=SampleTime
      link override Model/steam turbine/Stage 3/Stage3/Stage3/Model/Delay_x: SampleTime=SampleTime
      link override Model/steam turbine/Stage 3/Stage3/Stage3/Out: SampleTime=SampleTime
      link override Model/steam turbine/Stage 4/Constant1: SampleTime=SampleTime
      link override Model/steam turbine/Stage 4/Stage4/Stage4: Ts=SampleTime
      link override Model/steam turbine/Stage 4/Stage4/Stage4/In: SampleTime=SampleTime
      link override Model/steam turbine/Stage 4/Stage4/Stage4/Model/Delay_x: SampleTime=SampleTime
      link override Model/steam turbine/Stage 4/Stage4/Stage4/Out: SampleTime=SampleTime
      settings: LibrarySourceBlock=|
      | sps_lib/Electrical Machines/Synchronous Machine Control/Steam Turbine
      | and Governor
  Sum2 : Sum  InputSameDT=on  SaturateOnIntegerOverflow=on  SampleTime=SampleTime  OutDataTypeStr=Inherit: Same as first input
  Terminator : Terminator
  Terminator1 : Terminator
  Terminator2 : Terminator
  wref : Constant  SampleTime=SampleTime
  Pm1 : Outport  SampleTime=SampleTime  InitialOutput=0
  Vf1 : Outport  Port=2  SampleTime=SampleTime  InitialOutput=0
  tag scope: EFD1=global, Pe1=global, Q1=global, Vt1=global, d_theta1=global, pss1=global, theta1=global, w1=global
  wires:
  Bus Selector/7 -> EXCITATION1/3, Real-Imag to Complex/2  "<Stator voltage  vq (pu)>"
  wref/1 -> STG1/1
  Pref1/1 -> STG1/2
  m/1 -> Bus Selector/1
  Vref1/1 -> EXCITATION1/1
  EXCITATION1/1 -> Vf1/1, [EFD1]
  Real-Imag to Complex/1 -> [Vt1]
  Bus Selector/5 -> [theta1]  "<Rotor mechanical angle  theta (deg)>"
  Bus Selector/6 -> Real-Imag to Complex/1, EXCITATION1/2  "<Stator voltage  vd (pu)>"
  STG1/3 -> Terminator/1
  STG1/4 -> Pm1/1, Pm1_G1_log/1
  STG1/2 -> Terminator1/1
  STG1/1 -> Terminator2/1
  Bus Selector/1 -> [w1], STG1/3  "<Rotor speed  wm  (pu)>"
  Bus Selector/2 -> [d_theta1], STG1/4  "<Rotor angle deviation  d_theta (rad)>"
  Bus Selector/3 -> [Pe1]  "<Electrical power  Pe (pu)>"
  Bus Selector/8 -> [Q1]  "<Output reactive power  Qeo (pu)>"
  PSS1/1 -> Sum2/1
  Sum2/1 -> Multiport Switch1/1
  PSS model4/1 -> Sum2/2
  Multi-Band Power System Stabilizer/1 -> Multiport Switch1/3
  PSS model3/1 -> Multiport Switch1/2
  Multiport Switch1/1 -> [pss1], EXCITATION1/4
  Bus Selector/4 -> Multi-Band Power System Stabilizer/1  "<Rotor speed deviation  dw (pu)>"
